simulink model "Increment_test"  (R2023a)
settings: Solver=ode4  StartTime=0.0  StopTime=100  FixedStep=0.001  RelTol=1e-3
libraries: checkpacklib x1
settings Model: Creator=james  LastModifiedBy=james

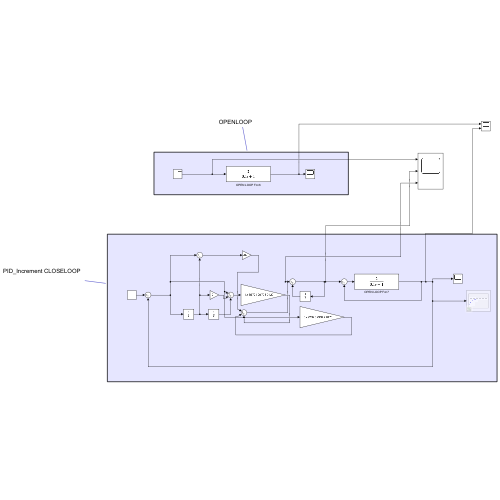
[thumbnail: Simulink's stored preview of the top-level diagram]
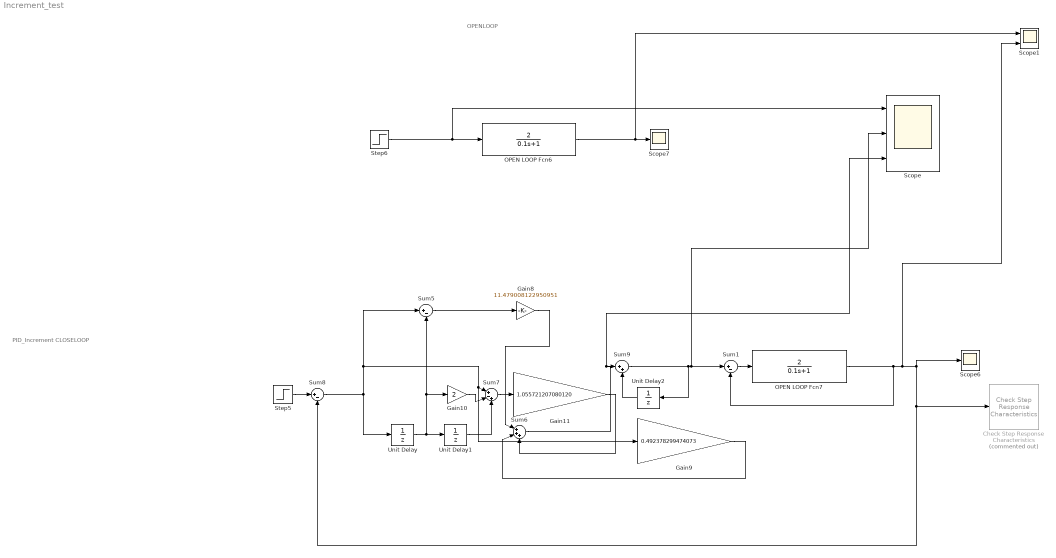
== system Increment_test ==
  note: PID_Increment CLOSELOOP
  note: OPENLOOP
  Check Step Response Characteristics : checkpacklib/Check Step Response  Characteristics  Commented=on  InstantiateOnLoad=on  enabled=on  stopWhenAssertionFail=off  export=off  ViewDlgPos=[100 199.666666666667 510 390]  OpenViewOnLoad=off  LaunchViewOnOpen=off  TimeUnits=seconds  EnableStepResponseBound=on  InitialValue=0  FinalValue=1  StepTime=0  RiseTime=5  PercentRise=80  SettlingTime=7  PercentSettling=1  PercentOvershoot=10  PercentUndershoot=1
      settings: LibrarySourceBlock=|
      | sdolib/Model Verification/Check Step Response
      | Characteristics
  Gain10 : Gain  Gain=2
  Gain11 : Gain  Gain=1.055721207080120
  Gain8 : Gain  Gain=11.479008122950951
  Gain9 : Gain  Gain=0.492378299474073
  OPEN LOOP Fcn6 : TransferFcn  Numerator=[2]  Denominator=[0.1 1]
  OPEN LOOP Fcn7 : TransferFcn  Numerator=[2]  Denominator=[0.1 1]
  Scope : Scope  NumInputPorts=3
  Scope1 : Scope  NumInputPorts=2
  Scope6 : Scope
  Scope7 : Scope
  Step5 : Step  SampleTime=0
  Step6 : Step  SampleTime=0
  Sum1 : Sum  Inputs=|+-
  Sum5 : Sum  Inputs=|+-
  Sum6 : Sum  Inputs=|+++
  Sum7 : Sum  Inputs=|+-+
  Sum8 : Sum  Inputs=|+-
  Sum9 : Sum  Inputs=|++
  Unit Delay : UnitDelay  SampleTime=0.001  HasFrameUpgradeWarning=on
  Unit Delay1 : UnitDelay  SampleTime=0.001  HasFrameUpgradeWarning=on
  Unit Delay2 : UnitDelay  SampleTime=0.001  HasFrameUpgradeWarning=on
  wires:
  Unit Delay2/1 -> Sum9/2
  Sum9/1 -> Sum1/1, Scope/2, Unit Delay2/1
  OPEN LOOP Fcn7/1 -> Sum1/2, Scope1/2, Scope6/1, Sum8/2, Check Step Response Characteristics/1
  Gain8/1 -> Sum6/1
  Gain9/1 -> Sum6/2
  Sum5/1 -> Gain8/1
  Unit Delay/1 -> Gain10/1, Sum5/2, Unit Delay1/1
  Sum8/1 -> Sum7/1, Gain9/1, Sum5/1, Unit Delay/1
  Gain10/1 -> Sum7/2
  Gain11/1 -> Sum6/3
  Step5/1 -> Sum8/1
  Unit Delay1/1 -> Sum7/3
  Sum1/1 -> OPEN LOOP Fcn7/1
  Sum7/1 -> Gain11/1
  Sum6/1 -> Scope/3, Sum9/1
  OPEN LOOP Fcn6/1 -> Scope1/1, Scope7/1
  Step6/1 -> Scope/1, OPEN LOOP Fcn6/1
